simulink model "Grid_ModelSimVSGConB"  (R2025b)
settings: Solver=daessc  StartTime=0.0  StopTime=10  MaxStep=1e-5  RelTol=1e-3
InitFcn:
  | Grid_ModelSimV1
values from neighbouring files (symbols this model uses):
  a = 0.5    [Grid_ModelSimV1.m]
  b = (beta*gamma)/(beta + gamma - a)    [Grid_ModelSimV1.m]
  c = (beta + gamma - a)/mp    [Grid_ModelSimV1.m]
  D1 = Moh_Dp/Moh_Sbase    (= 0.2546)    [Grid_ModelSimV1.m]
  D2 = 0.4    [Grid_ModelSimV1.m]
  delta1_0 = delta1PCC0 + atan2(      P12_0*X1/V1PCCmag0,      V1PCCmag0 + Q12_0*X1/V1PCCmag0 )    [Grid_ModelSimV1.m]
  delta2_0 = delta2PCC0 + atan2(      Pm2_0*X2/V2PCCmag0,      V2PCCmag0 + Q21_0*X2/V2PCCmag0 )    [Grid_ModelSimV1.m]
  Dw1_0 = 0    [Grid_ModelSimV1.m]
  Dw2_0 = 0    [Grid_ModelSimV1.m]
  E2_0 = hypot(      Pm2_0*X2/V2PCCmag0,      V2PCCmag0 + Q21_0*X2/V2PCCmag0 )    [Grid_ModelSimV1.m]
  H1 = J*omega_nom^2/2    (= 39.9916370332)    [Grid_ModelSimV1.m]
  H2 = 12    [Grid_ModelSimV1.m]
  Imax = 1.20    (= 1.2)    [Grid_ModelSimV1.m]
  J = Moh_J/Moh_Sbase    (= 0.0008104)    [Grid_ModelSimV1.m]
  Ki = 0.5    [Grid_ModelSimV1.m]
  Kiq = Moh_Kiq*Moh_Sbase/Moh_Vbase    [Grid_ModelSimV1.m]
  Lf = 1e-3    (= 0.001)    [Grid_ModelSimV1.m]
  LimitEnable = 1    [Grid_ModelSimV1.m]
  Ls = Xs/ws    [Grid_ModelSimV1.m]
  Ls_line = Xs_line/ws    [Grid_ModelSimV1.m]
  nq = Moh_nq*Moh_Sbase/Moh_Vbase    [Grid_ModelSimV1.m]
  omega_nom = ws    (= 314.159265359)    [Grid_ModelSimV1.m]
  Pload_0 = P12_0    (= 1)    [Grid_ModelSimV1.m]
  Qref = 0.0    (= 0)    [Grid_ModelSimV1.m]
  Rf = 1.0    (= 1)    [Grid_ModelSimV1.m]
  RLFault = 0    [Grid_ModelSimV1.m]
  Rs = Zs_mag/sqrt(1 + XR_grid^2)    [Grid_ModelSimV1.m]
  Rs_line = GridLineFraction*Rs    [Grid_ModelSimV1.m]
  SolidFault = 0    [Grid_ModelSimV1.m]
  ws = 2*pi*f    (= 314.159265359)    [Grid_ModelSimV1.m]
  X1 = Xtf_src_total_pu    (= 0.15)    [Grid_ModelSimV1.m]
libraries: nesl_utility x87, ee_lib x78, fl_lib x40, eePowerMeasurement x7
(part 2 of 6)

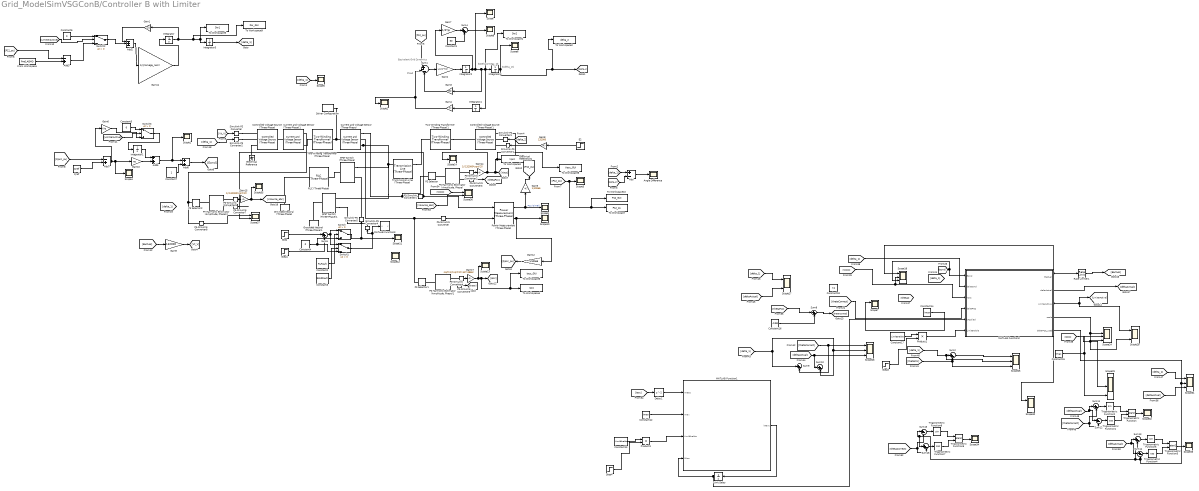
== system Grid_ModelSimVSGConB/Controller B with Limiter ==
  note: Pload
  note: Equivalent Grid Dynamics
  note: $\Delta\omega_2$
  note: $\delta_2$
  Add : Sum  Inputs=+-
  Add2 : Sum  Inputs=-+-
  Add3 : Sum  Inputs=-+
  Add5 : Sum
  Add6 : Sum
  Add7 : Sum  Inputs=-+
  Angle Difference : Scope
      settings: ActiveDisplayYMinimum=-0.016064112953822623  ActiveDisplayYMaximum=0.3934233708821307  DataLoggingVariableName=ScopeData11
  Constant1 : Constant  Value=50
  Constant12 : Constant  Value=Imax
  Constant13 : Constant  Value=LimitEnable
  Constant14 : Constant  Value=Imax
  Constant15 : Constant  Value=Imax
  Constant16 : Constant  Value=-0.58
  Constant17 : Constant  Value=LimitEnable
  Constant18 : Constant  Value=X1
  Constant2 : Constant  Value=RLFault
  Constant3 : Constant  Value=SolidFault
  Constant4 : Constant  Value=0
  Constant5 : Constant  Value=0
  Constant6 : Constant  Value=0
  Constant7 : Constant
  Controlled Voltage Source (Three-Phase) : ee_lib/Sources/Controlled Voltage Source (Three-Phase)  input_option=ee.enum.inputType.singleFreqAC  FRated=50 Hz
      settings: InternalSimscapePortConfiguration="{\"Bottom\":[],\"Left\":[{\"id\":\"Vt\",\"label\":\"Vt\",\"type\":\"input\"},{\"id\":\"ph\",\"label\":\"ph\",\"type\":\"input\"},{\"id\":\"n\",\"label\":\"n\",\"type\":\"foundation.electrical.electrical\"}],\"Right\":[{\"id\":\"N\",\"label\":\"~\",\"type\":\"foundation.electrical.three_phase\"}],\"Top\":[]}"
  Controlled Voltage Source (Three-Phase)1 : ee_lib/Sources/Controlled Voltage Source (Three-Phase)  input_option=ee.enum.inputType.singleFreqAC  FRated=50 Hz
      settings: InternalSimscapePortConfiguration="{\"Bottom\":[],\"Left\":[{\"id\":\"Vt\",\"label\":\"Vt\",\"type\":\"input\"},{\"id\":\"ph\",\"label\":\"ph\",\"type\":\"input\"},{\"id\":\"n\",\"label\":\"n\",\"type\":\"foundation.electrical.electrical\"}],\"Right\":[{\"id\":\"N\",\"label\":\"~\",\"type\":\"foundation.electrical.three_phase\"}],\"Top\":[]}"
  Current and Voltage Sensor (Three-Phase) : ee_lib/Sensors & Transducers/Current and Voltage Sensor (Three-Phase)  vMeasurementType=ee.enum.vmeasurement.ll  outputUnit=ee.enum.unit.si  SRated=100e6 A*V  VRated=24e3 V  I_specify=off  I_priority=None  I=[0, 0, 0] A  I_nominal_specify=off  I_nominal_value=1  I_nominal_unit=A  V_specify=off  V_priority=None  V=[0, 0, 0] V  V_nominal_specify=off  V_nominal_value=1  V_nominal_unit=V
      settings: InternalSimscapePortConfiguration="{\"Bottom\":[],\"Left\":[{\"id\":\"N1\",\"label\":\"~1\",\"type\":\"foundation.electrical.three_phase\"}],\"Right\":[{\"id\":\"V_output\",\"label\":\"V\",\"type\":\"output\"},{\"id\":\"I_output\",\"label\":\"I\",\"type\":\"output\"},{\"id\":\"N2\",\"label\":\"~2\",\"type\":\"foundation.electrical.three_phase\"}],\"Top\":[]}"
  Current and Voltage Sensor (Three-Phase)1 : ee_lib/Sensors & Transducers/Current and Voltage Sensor (Three-Phase)  vMeasurementType=ee.enum.vmeasurement.ll  outputUnit=ee.enum.unit.si  SRated=100e6 A*V  VRated=24e3 V  I_specify=off  I_priority=None  I=[0, 0, 0] A  I_nominal_specify=off  I_nominal_value=1  I_nominal_unit=A  V_specify=off  V_priority=None  V=[0, 0, 0] V  V_nominal_specify=off  V_nominal_value=1  V_nominal_unit=V
      settings: InternalSimscapePortConfiguration="{\"Bottom\":[],\"Left\":[{\"id\":\"N1\",\"label\":\"~1\",\"type\":\"foundation.electrical.three_phase\"}],\"Right\":[{\"id\":\"V_output\",\"label\":\"V\",\"type\":\"output\"},{\"id\":\"I_output\",\"label\":\"I\",\"type\":\"output\"},{\"id\":\"N2\",\"label\":\"~2\",\"type\":\"foundation.electrical.three_phase\"}],\"Top\":[]}"
  Delay1 : Delay  InitialCondition=1  SampleTime=1e-4
  E2 : Step  Before=E2_0  After=E2_0  SampleTime=0
  Electrical Reference : fl_lib/Electrical/Electrical Elements/Electrical Reference
  Electrical Reference1 : fl_lib/Electrical/Electrical Elements/Electrical Reference
  From Workspace : FromWorkspace  VariableName=Pref_AEMO  Interpolate=off  OutputAfterFinalValue=Holding final value
  Gain1 : Gain  Gain=D1
  Gain10 : Gain  Gain=nq
  Gain11 : Gain  Gain=1/(J*omega_nom)
  Gain12 : Gain  Gain=1/100e6
  Gain13 : Gain  Gain=sqrt(3)/(sqrt(2)*437.3866)
  Gain14 : Gain  Gain=1/(132000*sqrt(2))
  Gain15 : Gain  Gain=1/(132000*sqrt(2))
  Gain2 : Gain  Gain=ws/(2*H2)
  Gain3 : Gain  Gain=D2
  Gain4 : Gain  Gain=Ki
  Gain5 : Gain  Gain=1/100e6
  Gain6 : Gain  Gain=Kiq
  Gain7 : Gain  Gain=1/2*pi
  Gain8 : Gain  Gain=132000
  Gain9 : Gain  Gain=132000
  Grounded Neutral (Three-Phase) : ee_lib/Connectors & References/Grounded Neutral (Three-Phase)
  Grounded Neutral (Three-Phase)1 : ee_lib/Connectors & References/Grounded Neutral (Three-Phase)
  Integrator : Integrator
  Integrator1 : Integrator
  Integrator2 : Integrator  InitialCondition=Dw2_0
  Integrator3 : Integrator  InitialCondition=delta2_0
  Integrator4 : Integrator  InitialCondition=Pload_0/Ki
  Integrator5 : Integrator
  MATLAB Function1 : MATLAB Function  TreatAsAtomicUnit=on
  MATLAB Function2 : MATLAB Function  TreatAsAtomicUnit=on
  MATLAB Function3 : MATLAB Function  TreatAsAtomicUnit=on
  "PS Harmonic Estimator (Amplitude, Phase)" : fl_lib/Physical Signals/Periodic Operators/PS Harmonic Estimator (Amplitude, Phase)  f0=50 Hz  n=1  amplMin=0.001 V
      settings: InternalSimscapePortConfiguration="{\"Bottom\":[],\"Left\":[{\"id\":\"I\",\"label\":\"I\",\"type\":\"input\"}],\"Right\":[{\"id\":\"A\",\"label\":\"A\",\"type\":\"output\"},{\"id\":\"Phi\",\"label\":\"Phi\",\"type\":\"output\"}],\"Top\":[]}"
  "PS Harmonic Estimator (Amplitude, Phase)1" : fl_lib/Physical Signals/Periodic Operators/PS Harmonic Estimator (Amplitude, Phase)  f0=50 Hz  n=1  amplMin=0.001 A
      settings: InternalSimscapePortConfiguration="{\"Bottom\":[],\"Left\":[{\"id\":\"I\",\"label\":\"I\",\"type\":\"input\"}],\"Right\":[{\"id\":\"A\",\"label\":\"A\",\"type\":\"output\"},{\"id\":\"Phi\",\"label\":\"Phi\",\"type\":\"output\"}],\"Top\":[]}"
  "PS Harmonic Estimator (Amplitude, Phase)2" : fl_lib/Physical Signals/Periodic Operators/PS Harmonic Estimator (Amplitude, Phase)  f0=50 Hz  n=1  amplMin=0.001 V
      settings: InternalSimscapePortConfiguration="{\"Bottom\":[],\"Left\":[{\"id\":\"I\",\"label\":\"I\",\"type\":\"input\"}],\"Right\":[{\"id\":\"A\",\"label\":\"A\",\"type\":\"output\"},{\"id\":\"Phi\",\"label\":\"Phi\",\"type\":\"output\"}],\"Top\":[]}"
  PS Selector : fl_lib/Physical Signals/Nonlinear Operators/PS Selector  ix=1
      settings: InternalSimscapePortConfiguration="{\"Bottom\":[],\"Left\":[{\"id\":\"I\",\"label\":\"\",\"type\":\"input\"}],\"Right\":[{\"id\":\"O\",\"label\":\"\",\"type\":\"output\"}],\"Top\":[]}"
  PS Selector1 : fl_lib/Physical Signals/Nonlinear Operators/PS Selector  ix=1
      settings: InternalSimscapePortConfiguration="{\"Bottom\":[],\"Left\":[{\"id\":\"I\",\"label\":\"\",\"type\":\"input\"}],\"Right\":[{\"id\":\"O\",\"label\":\"\",\"type\":\"output\"}],\"Top\":[]}"
  PS Selector2 : fl_lib/Physical Signals/Nonlinear Operators/PS Selector  ix=1
      settings: InternalSimscapePortConfiguration="{\"Bottom\":[],\"Left\":[{\"id\":\"I\",\"label\":\"\",\"type\":\"input\"}],\"Right\":[{\"id\":\"O\",\"label\":\"\",\"type\":\"output\"}],\"Top\":[]}"
  PS-Simulink Converter{,1..8} (9 alike) : nesl_utility/PS-Simulink Converter  PhysicalDomain=network_engine_domain  SubClassName=ps_output  LeftPortType=input  RightPortType=output  PseudoPeriodic=off  Frequencies=[]  VectorFormat=inherit  Unit=inherit  AffineConversion=off
  Power Measurement (Three-Phase) : eePowerMeasurement/Power Measurement (Three-Phase)  LabelModeActiveChoice=Continuous  F=50  K=1  Seq=Positive  Ts=0
  Product1 : Product
  Product3 : Product
  Qref : Constant  Value=Qref
  RLC (Three-Phase) : ee_lib/Passive/RLC Assemblies/RLC (Three-Phase)  port_option=ee.enum.threePhasePort.composite  component_structure=ee.enum.rlc.structure.SeriesRL  R=Rf Ohm  L=Lf H  C=1e-6 F  R_parasitic=0 Ohm  G_parasitic=0 1/Ohm  IL_specify=off  IL_priority=High  IL=[0, 0, 0] A  IL_nominal_specify=off  IL_nominal_value=1  IL_nominal_unit=A  VC_specify=off  VC_priority=High  VC=[0, 0, 0] V  VC_nominal_specify=off  VC_nominal_value=1  VC_nominal_unit=V
      settings: InternalSimscapePortConfiguration="{\"Bottom\":[],\"Left\":[{\"id\":\"N1\",\"label\":\"~1\",\"type\":\"foundation.electrical.three_phase\"}],\"Right\":[{\"id\":\"N2\",\"label\":\"~2\",\"type\":\"foundation.electrical.three_phase\"}],\"Top\":[]}"
  Rate Limiter1 : RateLimiter  RisingSlewLimit=5  FallingSlewLimit=-1000  SampleTimeMode=inherited
  SPST Switch (Three-Phase) : ee_lib/Switches & Breakers/SPST Switch (Three-Phase)  R_closed=0.001 Ohm  G_open=1e-6 1/Ohm  threshold=0.5 V  i_vT_specify=off  i_vT_priority=None  i_vT=0 A  i_vT_nominal_specify=off  i_vT_nominal_value=1  i_vT_nominal_unit=A  I_specify=off  I_priority=None  I=[0, 0, 0] A  I_nominal_specify=off  I_nominal_value=1  I_nominal_unit=A  V_specify=off  V_priority=None  V=[0, 0, 0] V  V_nominal_specify=off  V_nominal_value=1  V_nominal_unit=V  i_a_specify=off  i_a_priority=None  i_a=0 A  i_a_nominal_specify=off  i_a_nominal_value=1  i_a_nominal_unit=A  v_a_specify=off  v_a_priority=None  v_a=0 V  v_a_nominal_specify=off  v_a_nominal_value=1  v_a_nominal_unit=V  i_b_specify=off  i_b_priority=None  i_b=0 A  i_b_nominal_specify=off  i_b_nominal_value=1  i_b_nominal_unit=A  v_b_specify=off  v_b_priority=None  v_b=0 V  v_b_nominal_specify=off  v_b_nominal_value=1  v_b_nominal_unit=V  i_c_specify=off  i_c_priority=None  i_c=0 A  i_c_nominal_specify=off  i_c_nominal_value=1  i_c_nominal_unit=A  v_c_specify=off  v_c_priority=None  v_c=0 V  v_c_nominal_specify=off  v_c_nominal_value=1  v_c_nominal_unit=V
      settings: InternalSimscapePortConfiguration="{\"Bottom\":[],\"Left\":[{\"id\":\"vT\",\"label\":\"vT\",\"type\":\"input\"},{\"id\":\"N1\",\"label\":\"~1\",\"type\":\"foundation.electrical.three_phase\"}],\"Right\":[{\"id\":\"N2\",\"label\":\"~2\",\"type\":\"foundation.electrical.three_phase\"}],\"Top\":[]}"
  SPST Switch (Three-Phase)1 : ee_lib/Switches & Breakers/SPST Switch (Three-Phase)  R_closed=0.001 Ohm  G_open=1e-6 1/Ohm  threshold=0.5 V  i_vT_specify=off  i_vT_priority=None  i_vT=0 A  i_vT_nominal_specify=off  i_vT_nominal_value=1  i_vT_nominal_unit=A  I_specify=off  I_priority=None  I=[0, 0, 0] A  I_nominal_specify=off  I_nominal_value=1  I_nominal_unit=A  V_specify=off  V_priority=None  V=[0, 0, 0] V  V_nominal_specify=off  V_nominal_value=1  V_nominal_unit=V  i_a_specify=off  i_a_priority=None  i_a=0 A  i_a_nominal_specify=off  i_a_nominal_value=1  i_a_nominal_unit=A  v_a_specify=off  v_a_priority=None  v_a=0 V  v_a_nominal_specify=off  v_a_nominal_value=1  v_a_nominal_unit=V  i_b_specify=off  i_b_priority=None  i_b=0 A  i_b_nominal_specify=off  i_b_nominal_value=1  i_b_nominal_unit=A  v_b_specify=off  v_b_priority=None  v_b=0 V  v_b_nominal_specify=off  v_b_nominal_value=1  v_b_nominal_unit=V  i_c_specify=off  i_c_priority=None  i_c=0 A  i_c_nominal_specify=off  i_c_nominal_value=1  i_c_nominal_unit=A  v_c_specify=off  v_c_priority=None  v_c=0 V  v_c_nominal_specify=off  v_c_nominal_value=1  v_c_nominal_unit=V
      settings: InternalSimscapePortConfiguration="{\"Bottom\":[],\"Left\":[{\"id\":\"vT\",\"label\":\"vT\",\"type\":\"input\"},{\"id\":\"N1\",\"label\":\"~1\",\"type\":\"foundation.electrical.three_phase\"}],\"Right\":[{\"id\":\"N2\",\"label\":\"~2\",\"type\":\"foundation.electrical.three_phase\"}],\"Top\":[]}"
  Scope{,1..6,8..14,32..35} (18 alike) : Scope
      Scope1 settings: ActiveDisplayYMinimum=-0.05189  ActiveDisplayYMaximum=0.00577  DataLoggingVariableName=ScopeData14
      Scope10 settings: ActiveDisplayYMinimum=-7.0875379074731711E+6  ActiveDisplayYMaximum=3.5866343126415364E+7  DataLoggingVariableName=ScopeData10
      Scope11 settings: ActiveDisplayYMinimum=-1  ActiveDisplayYMaximum=1  DataLoggingVariableName=ScopeData12
      Scope12 settings: ActiveDisplayYMinimum=-1  ActiveDisplayYMaximum=1  DataLoggingVariableName=ScopeData13
      Scope13 settings: ActiveDisplayYMinimum=-1.0313612715858387  ActiveDisplayYMaximum=9.28225144427255  DataLoggingVariableName=ScopeData21
      Scope14 settings: ActiveDisplayYMinimum=-2.5658886223026931  ActiveDisplayYMaximum=3.94553749363296  DataLoggingVariableName=ScopeData24
      Scope2 settings: ActiveDisplayYMinimum=-1.1623447136135812  ActiveDisplayYMaximum=1.3781315704633705  DataLoggingVariableName=ScopeData2
      Scope3 settings: ActiveDisplayYMinimum=-0.75357948603241187  ActiveDisplayYMaximum=1.838037306832903  DataLoggingVariableName=ScopeData3
      Scope32 settings: ActiveDisplayYMinimum=-3.9269892876580919  ActiveDisplayYMaximum=3.9269891159141448  DataLoggingVariableName=ScopeData42
      Scope33 settings: ActiveDisplayYMinimum=-1  ActiveDisplayYMaximum=1  DataLoggingVariableName=ScopeData43
      Scope34 settings: ActiveDisplayYMinimum=-1.4401977699145856  ActiveDisplayYMaximum=2.6200072427590877  DataLoggingVariableName=ScopeData44
      Scope35 settings: ActiveDisplayYMinimum=-2.5658886223026931  ActiveDisplayYMaximum=3.94553749363296  DataLoggingVariableName=ScopeData45
      Scope4 settings: ActiveDisplayYMinimum=-1.22917  ActiveDisplayYMaximum=1.0625  DataLoggingVariableName=ScopeData15
      Scope5 settings: ActiveDisplayYMinimum=-0.5315157226665419  ActiveDisplayYMaximum=2.1795261958257051  DataLoggingVariableName=ScopeData5
      Scope6 settings: DataLoggingVariableName=ScopeData6
      Scope8 settings: ActiveDisplayYMinimum=49.92788610274394  ActiveDisplayYMaximum=50.170097472488152  DataLoggingVariableName=ScopeData8
      Scope9 settings: ActiveDisplayYMinimum=-1.4766113788136218E+7  ActiveDisplayYMaximum=1.3289502409322599E+8  DataLoggingVariableName=ScopeData9
  Scope{18,25..26,29,31} (5 alike) : Scope  NumInputPorts=3
      Scope18 settings: ActiveDisplayYMinimum=-0.12862546618818504  ActiveDisplayYMaximum=1.1576291956936657  DataLoggingVariableName=ScopeData16
      Scope25 settings: ActiveDisplayYMinimum=-2.6035343832796971  ActiveDisplayYMaximum=9.8526279409331341  DataLoggingVariableName=ScopeData34
      Scope26 settings: ActiveDisplayYMinimum=-2.7720251649113785  ActiveDisplayYMaximum=1.647845241487004  DataLoggingVariableName=ScopeData35
      Scope29 settings: ActiveDisplayYMinimum=-0.5707391589619073  ActiveDisplayYMaximum=5.1366524306571666  DataLoggingVariableName=ScopeData38
      Scope31 settings: ActiveDisplayYMinimum=-2.7504004579249388  ActiveDisplayYMaximum=0.52931298913436242  DataLoggingVariableName=ScopeData41
  Scope24 : Scope  NumInputPorts=4
      settings: ActiveDisplayYMinimum=-0.14999999999999997  ActiveDisplayYMaximum=1.3499999999999999  DataLoggingVariableName=ScopeData19
  Scope{7,27..28,30,36..37} (6 alike) : Scope  NumInputPorts=2
      Scope27 settings: ActiveDisplayYMinimum=-3.7225747393161841  ActiveDisplayYMaximum=4.13168438536474  DataLoggingVariableName=ScopeData36
      Scope28 settings: ActiveDisplayYMinimum=-0.12499999999999997  ActiveDisplayYMaximum=1.125  DataLoggingVariableName=ScopeData37
      Scope30 settings: ActiveDisplayYMinimum=-0.12499999999999997  ActiveDisplayYMaximum=1.125  DataLoggingVariableName=ScopeData40
      Scope36 settings: ActiveDisplayYMinimum=-0.12862548717403666  ActiveDisplayYMaximum=1.1576293845663301  DataLoggingVariableName=ScopeData46
      Scope37 settings: ActiveDisplayYMinimum=-5.8136309150621951E+7  ActiveDisplayYMaximum=7.4558695125245631E+7  DataLoggingVariableName=ScopeData47
      Scope7 settings: ActiveDisplayYMinimum=-1.1863011737345548  ActiveDisplayYMaximum=10.676710563610996  DataLoggingVariableName=ScopeData39
  Simulink-PS Converter{,1..5} (6 alike) : nesl_utility/Simulink-PS Converter  PhysicalDomain=network_engine_domain  SubClassName=ps_input  LeftPortType=input  RightPortType=output  PseudoPeriodic=off  Frequencies=[]  NoiseDistribution=none  NoiseParameters=[]  Unit=1  AffineConversion=off  FilteringAndDerivatives=provide  SimscapeFilterOrder=1  InputFilterTimeConstant=0.001  UdotUserProvided=0
  Solver Configuration : nesl_utility/Solver Configuration  PhysicalDomain=network_engine_domain  SubClassName=solver  LeftPortType=input  RightPortType=generic  Tones=[]  Harmonics=[]  SimulateNoise=off  Profile=off  UseLocalSampling=off  EnableSwitchedLinearOptims=on  FrequencyDomain=off  UseCCode=off  RelTol=0.001  AbsTol=0.001  MinStep=1e-09  ToWorkspace=off  RevertToSquareIcSolve=off  NumHomotopyIterations=100  PhasorMode=off  PhasorModeNumHarmonics=1  ConsistencySolver=NEWTON_XTOL_AFTER_FTOL  IndexReductionMethod=DerivativeReplacement  DoDC=off  ResidualTolerance=1e-09  ConsistencyTolSource=GLOBAL  ConsistencyAbsTol=0.001  ConsistencyRelTol=0.001  ConsistencyTolFactor=0.001  UseLocalSolver=off  LocalSolverChoice=NE_BACKWARD_EULER_ADVANCER  ResolveIndetEquations=on  FunctionEvalNumThread=1  LocalSolverSampleTime=0.001  DoFixedCost=off  MaxNonlinIter=3  MaxModeIter=2  ComputeImpulses=off  ImpulseIterations=2  LinearAlgebra=auto  LinearAlgebraNumThread=0  EquationFormulation=NE_TIME_EF  DelaysMemoryBudget=1024  AutomaticFiltering=on  FilteringTimeConstant=0.001  PartitionStorageMethod=AS_NEEDED  PartitionMemoryBudget=1024  PartitionMethod=ROBUST  MultibodyUseLocalSolver=off  MultibodyLocalSolverChoice=ODE1  MultibodyLocalSolverSampleTime=0.001
  Step : Step  Time=5  SampleTime=0
  Step1 : Step  Time=5.43  After=-1  SampleTime=0
  Step3 : Step  Time=3  SampleTime=0
  Step4 : Step  Time=3  SampleTime=0
  Sum1 : Sum  Inputs=|+|-|-
  Sum{2,9..16} (9 alike) : Sum  Inputs=|+-
  Sum4 : Sum  Inputs=|++
  Sum6 : Sum  Inputs=|++
  Sum8 : Sum  Inputs=|++
  Switch{,1..3} (4 alike) : Switch  Criteria=u2 > Threshold  SaturateOnIntegerOverflow=off  InputSameDT=off
  To Workspace : ToWorkspace  VariableName=P12_pu  SaveFormat=Timeseries  SampleTime=-1
  To Workspace1 : ToWorkspace  VariableName=Dw2  SaveFormat=Timeseries  SampleTime=-1
  To Workspace10 : ToWorkspace  VariableName=P12_GUI  SaveFormat=Timeseries  SampleTime=-1
  To Workspace2 : ToWorkspace  VariableName=delta_2  SaveFormat=Timeseries  SampleTime=-1
  To Workspace3 : ToWorkspace  VariableName=Vpcc  SaveFormat=Timeseries  SampleTime=-1
  To Workspace4 : ToWorkspace  VariableName=Ipcc  SaveFormat=Timeseries  SampleTime=-1
  To Workspace5 : ToWorkspace  VariableName=Dw1  SaveFormat=Timeseries  SampleTime=-1
  To Workspace6 : ToWorkspace  VariableName=Ipcc_GUI  SaveFormat=Timeseries  SampleTime=-1
  To Workspace8 : ToWorkspace  VariableName=Vpcc_GUI  SaveFormat=Timeseries  SampleTime=-1
  To Workspace9 : ToWorkspace  VariableName=Dw_GUI  SaveFormat=Timeseries  SampleTime=-1
  Transmission Line (Three-Phase) : ee_lib/Passive/Lines/Transmission Line (Three-Phase)  length=1 km  freq=f Hz  R=Rs Ohm/km  L=Ls*1000 mH/km  M=0 mH/km  Cl=0.3 uF/km  Cg=0.1 uF/km  Rm=0 Ohm/km  ModelTwoSections=ee.enum.enable.no  N=1  InterfacePosition=0.5 km  N1sec=1  N2sec=1  Access_ground=ee.enum.enable.no  R_parasitic=1e-6 Ohm  G_parasitic=1e-6 1/Ohm
      settings: InternalSimscapePortConfiguration="{\"Bottom\":[],\"Left\":[{\"id\":\"N1\",\"label\":\"~1\",\"type\":\"foundation.electrical.three_phase\"},{\"id\":\"g1\",\"label\":\"g1\",\"type\":\"foundation.electrical.electrical\"}],\"Right\":[{\"id\":\"N2\",\"label\":\"~2\",\"type\":\"foundation.electrical.three_phase\"},{\"id\":\"g2\",\"label\":\"g2\",\"type\":\"foundation.electrical.electrical\"}],\"Top\":[]}"
  Trigonometric Function : Trigonometry  Operator=atan2
  Trigonometric Function1 : Trigonometry  Operator=cos
  Trigonometric Function2 : Trigonometry
  Trigonometric Function3 : Trigonometry  Operator=atan2
  Trigonometric Function4 : Trigonometry  Operator=cos
  Trigonometric Function5 : Trigonometry
  Trigonometric Function6 : Trigonometry  Operator=atan2
  Trigonometric Function7 : Trigonometry  Operator=cos
  Trigonometric Function8 : Trigonometry
  Two-Winding Transformer (Three-Phase) : ee_lib/Passive/Transformers/Two-Winding Transformer (Three-Phase)  SRated=100e6 A*V  FRated=50 Hz  Winding1Connection=ee.enum.windingconnection.Yg  VRated1=132000 V  Winding2Connection=ee.enum.windingconnection.Yg  VRated2=132000 V  CoreType=ee.enum.coretype.threelimb  pu_Rw1=0.001  pu_Rw2=0.001  leakage_reactance_option=ee.enum.transformer_leakage.include  pu_Xl1=0.075  pu_Xl2=0.075  magnetizing_resistance_option=ee.enum.transformer_magnetizingResistance.exclude  pu_Rm=500  magnetizing_reactance_option=ee.enum.transformer_magnetizingReactance.exclude  saturation_option=ee.enum.transformer_saturation.exclude  pu_Xm=500  current_data=[0, .002, 1, 2]  magnetic_flux_data=[0, 1.2, 1.5, 1.51]  pu_X0=0.5  i1_specify=off  i1_priority=None  i1=[0, 0, 0] A  i1_nominal_specify=off  i1_nominal_value=1  i1_nominal_unit=A  i2_specify=off  i2_priority=None  i2=[0, 0, 0] A  i2_nominal_specify=off  i2_nominal_value=1  i2_nominal_unit=A  phi_specify=off  phi_priority=None  phi=[0, 0, 0]  phi_nominal_specify=off  phi_nominal_value=1  phi_nominal_unit=1  power_dissipated_specify=off  power_dissipated_priority=None  power_dissipated=0 W  power_dissipated_nominal_specify=off  power_dissipated_nominal_value=1  power_dissipated_nominal_unit=W
      settings: InternalSimscapePortConfiguration="{\"Bottom\":[],\"Left\":[{\"id\":\"N1\",\"label\":\"~1\",\"type\":\"foundation.electrical.three_phase\"}],\"Right\":[{\"id\":\"N2\",\"label\":\"~2\",\"type\":\"foundation.electrical.three_phase\"}],\"Top\":[]}"
  Two-Winding Transformer (Three-Phase)1 : ee_lib/Passive/Transformers/Two-Winding Transformer (Three-Phase)  SRated=100e6 A*V  FRated=50 Hz  Winding1Connection=ee.enum.windingconnection.Y  VRated1=132000 V  Winding2Connection=ee.enum.windingconnection.Y  VRated2=132000 V  CoreType=ee.enum.coretype.threelimb  pu_Rw1=0.001  pu_Rw2=0.001  leakage_reactance_option=ee.enum.transformer_leakage.include  pu_Xl1=0.075  pu_Xl2=0.075  magnetizing_resistance_option=ee.enum.transformer_magnetizingResistance.exclude  pu_Rm=500  magnetizing_reactance_option=ee.enum.transformer_magnetizingReactance.exclude  saturation_option=ee.enum.transformer_saturation.exclude  pu_Xm=500  current_data=[0, .002, 1, 2]  magnetic_flux_data=[0, 1.2, 1.5, 1.51]  pu_X0=0.5  i1_specify=off  i1_priority=None  i1=[0, 0, 0] A  i1_nominal_specify=off  i1_nominal_value=1  i1_nominal_unit=A  i2_specify=off  i2_priority=None  i2=[0, 0, 0] A  i2_nominal_specify=off  i2_nominal_value=1  i2_nominal_unit=A  phi_specify=off  phi_priority=None  phi=[0, 0, 0]  phi_nominal_specify=off  phi_nominal_value=1  phi_nominal_unit=1  power_dissipated_specify=off  power_dissipated_priority=None  power_dissipated=0 W  power_dissipated_nominal_specify=off  power_dissipated_nominal_value=1  power_dissipated_nominal_unit=W
      settings: InternalSimscapePortConfiguration="{\"Bottom\":[],\"Left\":[{\"id\":\"N1\",\"label\":\"~1\",\"type\":\"foundation.electrical.three_phase\"}],\"Right\":[{\"id\":\"N2\",\"label\":\"~2\",\"type\":\"foundation.electrical.three_phase\"}],\"Top\":[]}"
  Unit Delay : UnitDelay  InitialCondition=1  SampleTime=1e-4  HasFrameUpgradeWarning=on
  wires:
  Switch/1 -> Simulink-PS Converter5/1, Scope11/1
  Step1/1 -> Sum6/2
  Constant4/1 -> Switch1/3, Switch/3
  [P12_pu] -> To Workspace10/1, To Workspace/1, Scope3/1
  Power Measurement (Three-Phase)/2 -> Scope10/1, Gain12/1
  Gain3/1 -> Sum1/3
  Gain5/1 -> [P12_pu]
  Sum6/1 -> Switch1/1, Switch/1
  Add/1 -> Angle Difference/1
  PS-Simulink Converter1/1 -> Scope37/2, Power Measurement (Three-Phase)/1
  Constant3/1 -> Switch1/2
  Gain8/1 -> Simulink-PS Converter1/1
  Sum1/1 -> Gain2/1
  [delta_2] -> Add/2
  E2/1 -> Gain8/1
  Integrator2/1 -> Gain7/1, Scope/1, Gain3/1, To Workspace1/1, Integrator4/1, Integrator3/1
  [Vt_V] -> Simulink-PS Converter/1
  PS-Simulink Converter/1 -> Power Measurement (Three-Phase)/2
  Integrator4/1 -> Gain4/1
  Integrator3/1 -> To Workspace2/1, [delta_2], Scope6/1
  Gain4/1 -> Scope2/1, Sum1/2
  Constant1/1 -> Sum4/2
  Gain12/1 -> [Qpcc_pu]
  Gain9/1 -> [Vt_V]
  Gain2/1 -> Integrator2/1
  [delta_2] -> Simulink-PS Converter3/1
  [delta_1] -> Scope5/1
  Sum4/1 -> Scope8/1
  Gain7/1 -> Sum4/1
  Power Measurement (Three-Phase)/1 -> Scope9/1, Gain5/1  "P12 (SimEl)"
  [delta_1] -> Add/1
  [P12_pu] -> Sum1/1
  Step/1 -> Sum6/1
  Switch1/1 -> Simulink-PS Converter4/1, MATLAB Function3/1(u)
  Constant2/1 -> Switch/2
  Add5/1 -> Scope1/1, Add6/1
  Constant5/1 -> Switch3/1
  Qref/1 -> Add7/2
  Gain10/1 -> Add5/2
  [Qpcc_pu] -> Add7/1
  Integrator1/1 -> Add5/1
  Constant7/1 -> Add6/2
  Add6/1 -> [Ecmd]
  Add7/1 -> Gain6/1, Scope4/1, Gain10/1
  Switch3/1 -> Integrator1/1
  Gain6/1 -> Switch3/3
  [LimiterActive] -> Switch3/2
  Add2/1 -> Gain11/1
  From Workspace/1 -> Add3/2
  [LimiterActive] -> Switch2/2
  [P12_pu] -> Add3/1
  Gain1/1 -> Add2/1
  Gain11/1 -> Integrator/1
  Integrator5/1 -> [delta_1]
  Integrator/1 -> To Workspace9/1, Integrator5/1, To Workspace5/1, Gain1/1
  Add3/1 -> Switch2/3
  Switch2/1 -> Add2/2
  Constant6/1 -> Switch2/1
  ? -> ?
  [Eactual] -> Gain9/1
  PS-Simulink Converter4/1 -> Gain13/1
  Gain13/1 -> To Workspace6/1, To Workspace4/1, [Ipcc], Scope13/1
  PS-Simulink Converter2/1 -> Gain14/1
  Gain14/1 -> Scope14/1, To Workspace8/1, To Workspace3/1, [Vpcc]
  PS-Simulink Converter3/1 -> [thetaPcc]
  PS-Simulink Converter5/1 -> [thetaI]
  [delta_1] -> Simulink-PS Converter2/1
  MATLAB Function1/1(kNext) -> Unit Delay/1
  [Ipcc] -> Delay1/1
  Delay1/1 -> MATLAB Function1/1(Imeas)
  Constant12/1 -> MATLAB Function1/2(Imax)
  Constant13/1 -> Product3/1
  Step4/1 -> Product3/2
  Product3/1 -> MATLAB Function1/3(LimitEnable)
  [thetaPcc] -> Scope25/3, Sum2/2
  [Vpcc] -> Scope18/2, MATLAB Function2/3(Vpcc)
  [thetaCorrect] -> Sum9/2, Scope26/1
  [deltaActual] -> Scope27/2
  [delta_1] -> Sum9/1, Sum10/2, Scope26/2
  [delta_1] -> MATLAB Function2/2(deltaCmd)
  MATLAB Function2/3(LimiterActive) -> Scope30/1, [LimiterActive], Scope28/1
  [Ipcc] -> Scope29/2, Scope24/4
  [thetaCorrect] -> MATLAB Function2/4(deltaPCC)
  Product1/1 -> MATLAB Function2/6(LimitEnable)
  Constant16/1 -> Sum8/2
  [thetaPcc] -> Sum8/1
  Constant14/1 -> Scope7/1
  MATLAB Function2/1(Eactual) -> Scope18/1, Rate Limiter1/1
  Step3/1 -> Product1/2
  MATLAB Function2/4(scale) -> Scope28/2, Scope24/2
  Sum2/1 -> Scope25/1
  [deltaActual] -> Sum10/1, Scope26/3
  Sum8/1 -> [thetaCorrect]
  Constant17/1 -> Product1/1
  [delta_1] -> Scope25/2, Sum2/1
  [delta_1] -> Scope27/1
  [Ecmd] -> Scope18/3, MATLAB Function2/1(Ecmd)
  [deltaActual] -> Scope31/3
  [delta_1] -> Scope31/1
  Unit Delay/1 -> MATLAB Function2/5(kApplied), MATLAB Function1/4(kPrev)
  [deltaActual] -> Sum12/1, Sum11/1
  [thetaCorrect] -> Sum12/2, Sum11/2
  Trigonometric Function/1 -> Scope32/1
  Sum12/1 -> Trigonometric Function1/1
  Sum11/1 -> Trigonometric Function2/1
  Trigonometric Function1/1 -> Trigonometric Function/2
  Trigonometric Function2/1 -> Trigonometric Function/1
  Trigonometric Function3/1 -> Scope33/1
  [deltaActual] -> Sum14/1, Sum13/1
  Constant15/1 -> Scope29/3, Scope24/3
  Sum13/1 -> Trigonometric Function5/1
  Trigonometric Function5/1 -> Trigonometric Function3/1
  Trigonometric Function4/1 -> Trigonometric Function3/2
  Sum14/1 -> Trigonometric Function4/1
  Trigonometric Function6/1 -> Scope34/1
  MATLAB Function2/5(deltaPCC_used) -> Sum13/2, Sum15/1, Sum16/1, Sum14/2, Scope31/2
  [thetaCorrect] -> Sum16/2, Sum15/2
  Sum15/1 -> Trigonometric Function8/1
  Trigonometric Function8/1 -> Trigonometric Function6/1
  Trigonometric Function7/1 -> Trigonometric Function6/2
  Sum16/1 -> Trigonometric Function7/1
  MATLAB Function2/2(deltaActual) -> [deltaActual]
  PS-Simulink Converter7/1 -> ?
  PS-Simulink Converter6/1 -> Gain15/1
  Gain15/1 -> Scope35/1, [Vsource_abc]
  [Vsource_abc] -> Scope36/2
  [Vpcc] -> Scope36/1
  PS-Simulink Converter8/1 -> Scope37/1
  Rate Limiter1/1 -> [Eactual]
  connections:
  Simulink-PS Converter1/RConn1 -- Controlled Voltage Source (Three-Phase)1/LConn1
  Current and Voltage Sensor (Three-Phase)/RConn1 -- PS Selector/LConn1 -- PS-Simulink Converter1/LConn1
  Simulink-PS Converter3/RConn1 -- Controlled Voltage Source (Three-Phase)1/LConn2
  SPST Switch (Three-Phase)1/LConn1 -- Simulink-PS Converter4/RConn1
  Grounded Neutral (Three-Phase)1/LConn1 -- SPST Switch (Three-Phase)1/RConn1
  Two-Winding Transformer (Three-Phase)1/RConn1 -- Controlled Voltage Source (Three-Phase)1/RConn1
  Electrical Reference/LConn1 -- Controlled Voltage Source (Three-Phase)/LConn3
  Transmission Line (Three-Phase)/RConn1 -- Two-Winding Transformer (Three-Phase)1/LConn1
  Current and Voltage Sensor (Three-Phase)/LConn1 -- Solver Configuration/RConn1 -- Two-Winding Transformer (Three-Phase)/RConn1
  Current and Voltage Sensor (Three-Phase)/RConn3 -- Transmission Line (Three-Phase)/LConn1 -- SPST Switch (Three-Phase)1/LConn2 -- SPST Switch (Three-Phase)/LConn2
  Grounded Neutral (Three-Phase)/LConn1 -- RLC (Three-Phase)/LConn1
  Simulink-PS Converter/RConn1 -- Controlled Voltage Source (Three-Phase)/LConn1
  PS-Simulink Converter/LConn1 -- PS Selector1/LConn1 -- Current and Voltage Sensor (Three-Phase)/RConn2
  Simulink-PS Converter2/RConn1 -- Controlled Voltage Source (Three-Phase)/LConn2
  Electrical Reference1/LConn1 -- Controlled Voltage Source (Three-Phase)1/LConn3
  SPST Switch (Three-Phase)/RConn1 -- RLC (Three-Phase)/RConn1
  Simulink-PS Converter5/RConn1 -- SPST Switch (Three-Phase)/LConn1
  PS-Simulink Converter4/LConn1 -- "PS Harmonic Estimator (Amplitude, Phase)1"/RConn1
  "PS Harmonic Estimator (Amplitude, Phase)1"/LConn1 -- PS Selector1/RConn1
  PS-Simulink Converter2/LConn1 -- "PS Harmonic Estimator (Amplitude, Phase)"/RConn1
  "PS Harmonic Estimator (Amplitude, Phase)"/LConn1 -- PS Selector/RConn1
  PS-Simulink Converter3/LConn1 -- "PS Harmonic Estimator (Amplitude, Phase)"/RConn2
  PS-Simulink Converter5/LConn1 -- "PS Harmonic Estimator (Amplitude, Phase)1"/RConn2
  Current and Voltage Sensor (Three-Phase)1/LConn1 -- Controlled Voltage Source (Three-Phase)/RConn1
  Current and Voltage Sensor (Three-Phase)1/RConn3 -- Two-Winding Transformer (Three-Phase)/LConn1
  PS-Simulink Converter7/LConn1 -- "PS Harmonic Estimator (Amplitude, Phase)2"/RConn2
  "PS Harmonic Estimator (Amplitude, Phase)2"/LConn1 -- PS Selector2/RConn1
  PS-Simulink Converter6/LConn1 -- "PS Harmonic Estimator (Amplitude, Phase)2"/RConn1
  PS Selector2/LConn1 -- PS-Simulink Converter8/LConn1 -- Current and Voltage Sensor (Three-Phase)1/RConn1
